simulink model "ex2"  (R2025a)
settings: Solver=VariableStepAuto  StartTime=0.0  StopTime=10.0  RelTol=1e-3
values from neighbouring files (symbols this model uses):
  K = 1/sqrt(2)    [sim2.m]
  L_M = 0.20    (= 0.2)    [sim2.m]
  L_sig = 0.025    [sim2.m]
  np = p    (= 2)    [sim2.m]
  R_R = 0.45    [sim2.m]
  R_s = 1    [sim2.m]
settings Model: Creator=dimit  LastModifiedBy=dimit

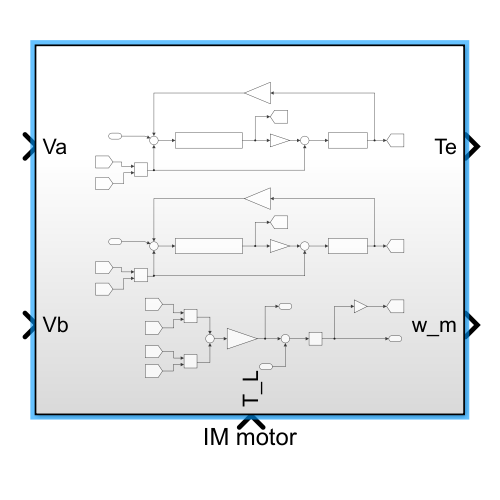
[thumbnail: Simulink's stored preview of the top-level diagram]
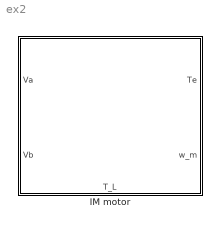
== system ex2 ==
  IM motor : Subsystem
      settings: PortSchema="{\"entries\":[{\"content\":{\"sides\":[{\"content\":{\"connectorIds\":[\"In1\",\"In2\"]},\"type\":\"ConnectorPlacement.EquallySpacedRectSide\",\"uuid\":\"51ce8d8d-f70a-4d74-9403-4a2ac025a85e\"},{\"content\":{\"connectorIds\":[\"Out1\",\"Out2\"],\"side\":\"RIGHT\"},\"type\":\"ConnectorPlacement.EquallySpacedRectSide\",\"uuid\":\"f6ddc1dd-9c6b-4de5-b80a-02e3b764712c\"},{\"content\":{\"side\":\"TOP\"},\"type\":\"ConnectorPlacement.EquallySpacedRectSide\",\"uuid\":\"73a75396-5d1b-4b35-87ea-52b4d5235389\"},{\"content\":{\"connectorIds\":[\"In3\"],\"side\":\"BOTTOM\"},\"type\":\"ConnectorPlacement.EquallySpacedRectSide\",\"uuid\":\"d9589691-4817-4dea-b8b9-f2a79ff709eb\"}]},\"type\":\"ConnectorPlacement.EquallySpacedConnector\",\"uuid\":\"567b54d3-078a-47f2-aacd-44aae6ed51ca\"}],\"packageUris\":[\"http://schema.mathworks.com/mf0/Connector/R2020b\"],\"version\":\"1.0\"}"

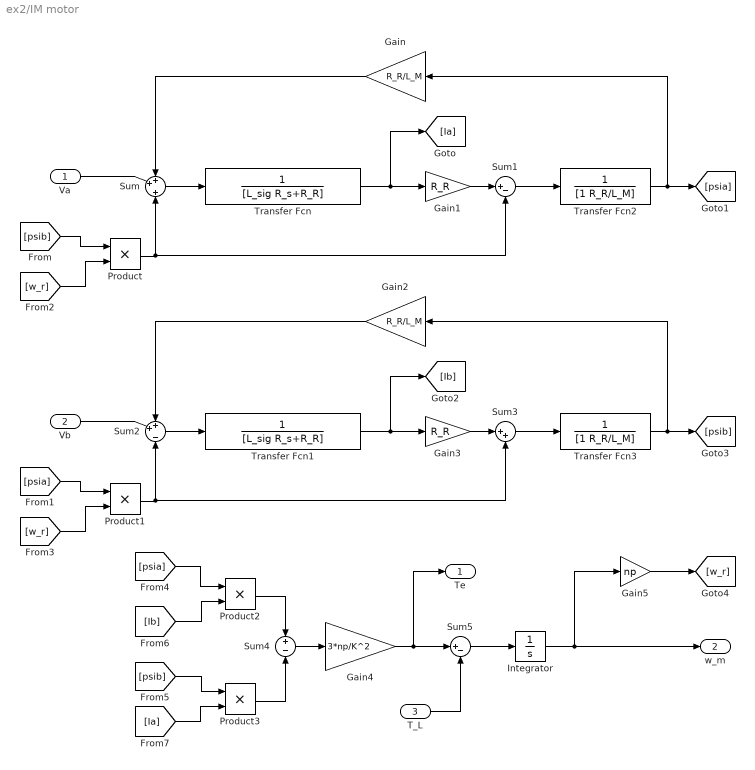
== system ex2/IM motor ==
  Va : Inport
  Vb : Inport  Port=2
  T_L : Inport  Port=3
  Gain : Gain  Gain=R_R/L_M
  Gain1 : Gain  Gain=R_R
  Gain2 : Gain  Gain=R_R/L_M
  Gain3 : Gain  Gain=R_R
  Gain4 : Gain  Gain=3*np/K^2
  Gain5 : Gain  Gain=np
  Integrator : Integrator
  Product{,1..3} (4 alike) : Product
  Sum : Sum  Inputs=++|+
  Sum1 : Sum  Inputs=|+-
  Sum2 : Sum  Inputs=++|-
  Sum3 : Sum  Inputs=|++
  Sum4 : Sum  Inputs=+|-
  Sum5 : Sum  Inputs=|+-
  Transfer Fcn : TransferFcn  Denominator=[L_sig R_s+R_R]
  Transfer Fcn1 : TransferFcn  Denominator=[L_sig R_s+R_R]
  Transfer Fcn2 : TransferFcn  Denominator=[1 R_R/L_M]
  Transfer Fcn3 : TransferFcn  Denominator=[1 R_R/L_M]
  Te : Outport
  w_m : Outport  Port=2
  wires:
  Sum/1 -> Transfer Fcn/1
  Transfer Fcn/1 -> [Ia], Gain1/1
  Transfer Fcn2/1 -> Gain/1, [psia]
  [psib] -> Product/1
  [w_r] -> Product/2
  Product/1 -> Sum1/2, Sum/3
  Gain1/1 -> Sum1/1
  Sum1/1 -> Transfer Fcn2/1
  Va/1 -> Sum/2
  Gain/1 -> Sum/1
  Vb/1 -> Sum2/2
  Transfer Fcn3/1 -> Gain2/1, [psib]
  Gain3/1 -> Sum3/1
  Product1/1 -> Sum3/2, Sum2/3
  Sum3/1 -> Transfer Fcn3/1
  [w_r] -> Product1/2
  Transfer Fcn1/1 -> [Ib], Gain3/1
  Sum2/1 -> Transfer Fcn1/1
  Gain2/1 -> Sum2/1
  [psia] -> Product1/1
  Gain4/1 -> Sum5/1, Te/1
  [psia] -> Product2/1
  [Ib] -> Product2/2
  Sum4/1 -> Gain4/1
  Product2/1 -> Sum4/1
  [psib] -> Product3/1
  [Ia] -> Product3/2
  Product3/1 -> Sum4/2
  T_L/1 -> Sum5/2
  Sum5/1 -> Integrator/1
  Integrator/1 -> Gain5/1, w_m/1
  Gain5/1 -> [w_r]
